simulink model "Lab5B_LinkageKinematics"  (R2026a)
settings: Solver=VariableStepAuto
values from neighbouring files (symbols this model uses):
  q0dot = q0dot_nom    [crank_piston_analysis.m]
  theta2 = deg2rad(120)    [crank_piston_analysis.m]
  theta2ddot = 0    [crank_piston_analysis.m]
  theta2dot = theta2dot_nom    (= -1.0471975512)    [crank_piston_analysis.m]
undefined symbols (not defined in the file or in its folder): q0
settings Model: Creator=jonbb  LastModifiedBy=jonbb

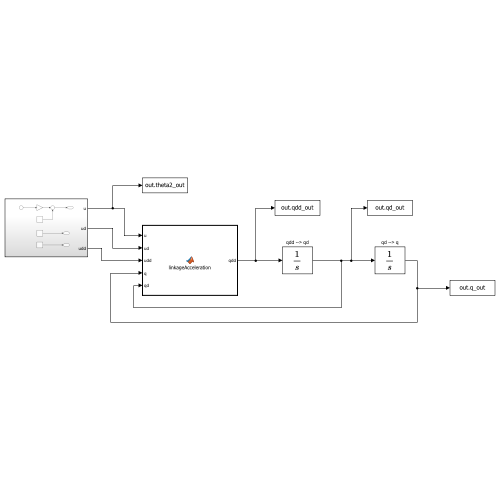
[thumbnail: Simulink's stored preview of the top-level diagram]
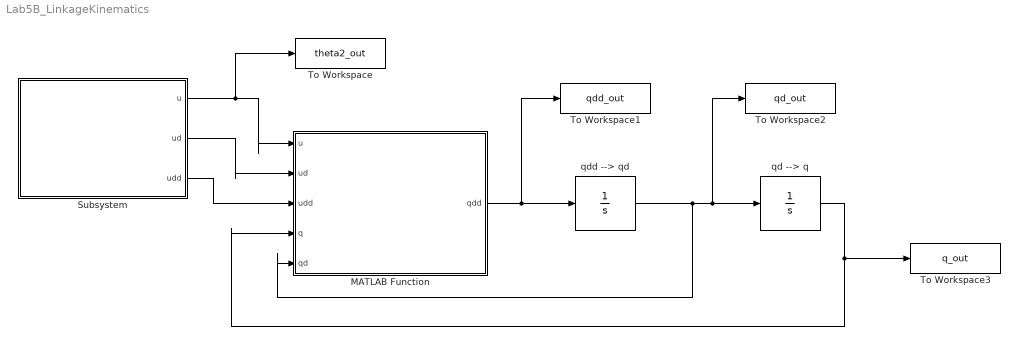
== system Lab5B_LinkageKinematics ==
  MATLAB Function : MATLAB Function  TreatAsAtomicUnit=on
  Subsystem : Subsystem
  To Workspace : ToWorkspace  VariableName=theta2_out  SampleTime=-1
  To Workspace1 : ToWorkspace  VariableName=qdd_out  SampleTime=-1
  To Workspace2 : ToWorkspace  VariableName=qd_out  SampleTime=-1
  To Workspace3 : ToWorkspace  VariableName=q_out  SampleTime=-1
  qd --> q : Integrator  InitialCondition=q0
  qdd --> qd : Integrator  InitialCondition=q0dot
  wires:
  qdd --> qd/1 -> MATLAB Function/5(qd), To Workspace2/1, qd --> q/1
  qd --> q/1 -> To Workspace3/1, MATLAB Function/4(q)
  Subsystem/1(u) -> To Workspace/1, MATLAB Function/1(u)
  Subsystem/2(ud) -> MATLAB Function/2(ud)
  Subsystem/3(udd) -> MATLAB Function/3(udd)
  MATLAB Function/1(qdd) -> To Workspace1/1, qdd --> qd/1

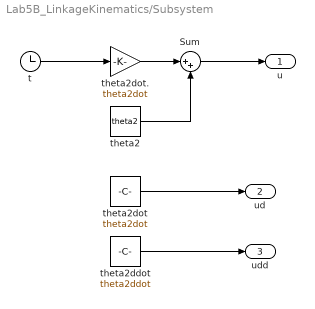
== system Lab5B_LinkageKinematics/Subsystem ==
  Sum : Sum  Inputs=|++
  t : Clock
  theta2 : Constant  Value=theta2
  theta2ddot : Constant  Value=theta2ddot
  theta2dot : Constant  Value=theta2dot
  theta2dot. : Gain  Gain=theta2dot
  u : Outport
  ud : Outport  Port=2
  udd : Outport  Port=3
  wires:
  t/1 -> theta2dot./1
  theta2/1 -> Sum/2
  theta2dot./1 -> Sum/1
  Sum/1 -> u/1
  theta2dot/1 -> ud/1
  theta2ddot/1 -> udd/1

== matlab function Lab5B_LinkageKinematics/MATLAB Function ==
  data: u input; qdd output; ud input; udd input; q input; qd input size=[2 1]; p parameter
function qdd = linkageAcceleration(u,ud,udd,q,qd,p)
% u = theta2, ud = theta2dot, udd = theta2ddot
% q = [r_ob; theta3], qd = [r_ob_dot, theta3dot]
theta3 = q(2);
theta3dot = qd(2);

J = [-1, -p.r_3*sin(theta3);
    0, p.r_3*cos(theta3)];

ba = [p.r_2*cos(u)*ud^2 + p.r_2*sin(u)*udd + p.r_3*cos(theta3)*theta3dot^2;
    p.r_2*sin(u)*ud^2 - p.r_2*cos(u)*udd + p.r_3*sin(theta3)*theta3dot^2];

qdd = J \ ba;

end
